simulink model "BO_SimulinkNonLinear"  (R2024b)
settings: Solver=VariableStepAuto  StartTime=0.0  StopTime=10.0  RelTol=1e-3
settings Model: Creator=dsagn  LastModifiedBy=dsagn
settings ConfigComp: CovMetricSettings=de  CovBoundaryAbsTol=1.0e-5

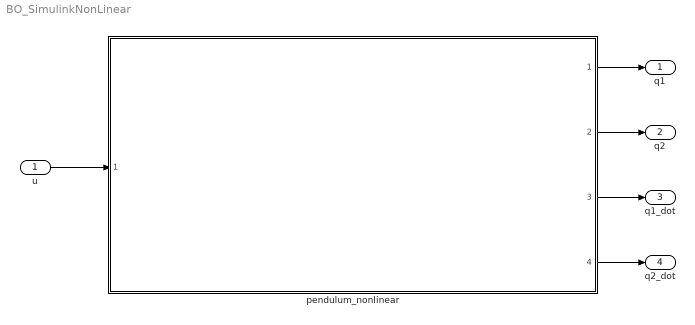
== system BO_SimulinkNonLinear ==
  "u " : Inport
  pendulum_nonlinear : Subsystem  ReferencedSubsystem=pendulum_nonlinear
  q1 : Outport  VectorParamsAs1DForOutWhenUnconnected=off
  "q2 " : Outport  Port=2  VectorParamsAs1DForOutWhenUnconnected=off
  q1_dot : Outport  Port=3  VectorParamsAs1DForOutWhenUnconnected=off
  q2_dot : Outport  Port=4  VectorParamsAs1DForOutWhenUnconnected=off
  wires:
  "u "/1 -> pendulum_nonlinear/1
  pendulum_nonlinear/1 -> q1/1
  pendulum_nonlinear/2 -> "q2 "/1
  pendulum_nonlinear/3 -> q1_dot/1
  pendulum_nonlinear/4 -> q2_dot/1
